simulink model "HarnessModel_CtrlEnv"  (R2026a)
settings: Solver=daessc  StopTime=100  AbsTol=1e-3
PreLoadFcn:
  | setupHarness_CtrlEnv
PostLoadFcn:
  | % Setup the model to use the "Simple" case
  | % for the Vehicle speed reference.
  | loadLUTData_VehSpdRef_Simple
  | set_param(bdroot, StopTime = "100")
  | set_param(bdroot + "/Controller and Environment/Vehicle speed reference", ...
  |     ReferencedSubsystem="VehSpdRef_LookupTable_refsub")
settings Model: Creator=isaacito  LastModifiedBy=isaacito
settings SimscapeCC: SimscapeNominalValues="[{\"value\":\"1\",\"unit\":\"A\"},{\"value\":\"1\",\"unit\":\"bar\"},{\"value\":\"1\",\"unit\":\"cm^2\"},{\"value\":\"1\",\"unit\":\"cm^3/s\"},{\"value\":\"1\",\"unit\":\"kJ/kg\"},{\"value\":\"1\",\"unit\":\"kW\"},{\"value\":\"1\",\"unit\":\"l\"},{\"value\":\"1\",\"unit\":\"N\"},{\"value\":\"1\",\"unit\":\"N*m\"},{\"value\":\"1\",\"unit\":\"V\"}]"  SimscapeLogSimulationStatistics=on  SimscapeLogLimitData=off  SimscapeLogDataHistory=5000.0

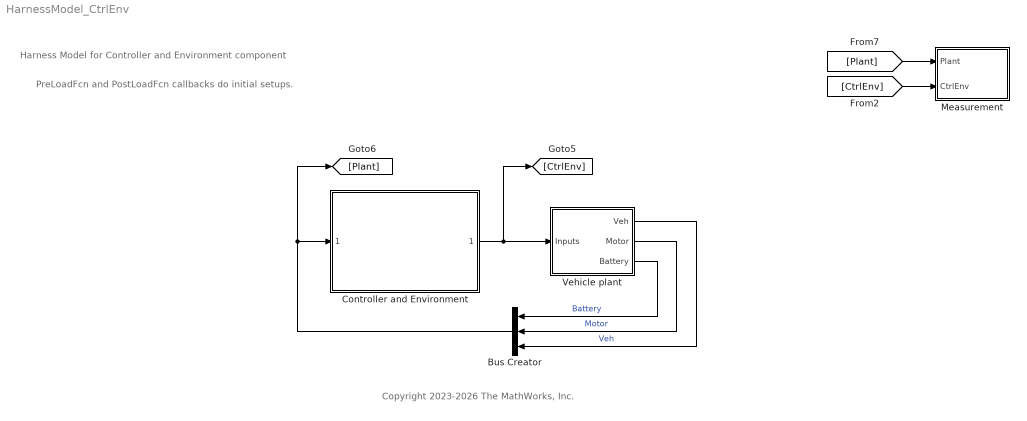
== system HarnessModel_CtrlEnv ==
  note: PreLoadFcn and PostLoadFcn callbacks do initial setups.
  note: Harness Model for Controller and Environment component
  note: Copyright 2023-2026 The MathWorks, Inc.
  Bus Creator : BusCreator  Inputs=3
  Controller and Environment : Subsystem  ReferencedSubsystem=CtrlEnv_Basic_refsub
      settings: OpenFcn=|
      | % Look under mask:
      | open_system(gcb, "force")
  Measurement : Subsystem
  Vehicle plant : Subsystem
  wires:
  [CtrlEnv] -> Measurement/2(CtrlEnv)
  [Plant] -> Measurement/1(Plant)
  Controller and Environment/1 -> Vehicle plant/1(Inputs), [CtrlEnv]
  Vehicle plant/1(Veh) -> Bus Creator/3  "Veh"
  Vehicle plant/2(Motor) -> Bus Creator/2  "Motor"
  Vehicle plant/3(Battery) -> Bus Creator/1  "Battery"
  Bus Creator/1 -> Controller and Environment/1, [Plant]

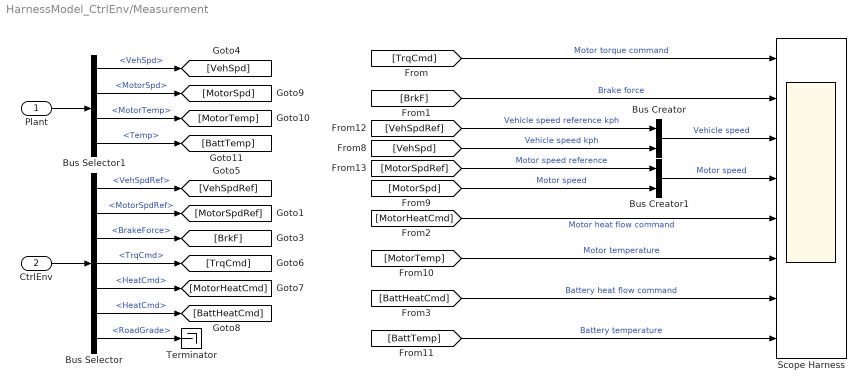
== system HarnessModel_CtrlEnv/Measurement ==
  Plant : Inport
  CtrlEnv : Inport  Port=2
  Bus Creator : BusCreator  Inputs=2
  Bus Creator1 : BusCreator  Inputs=2
  Bus Selector : BusSelector  OutputSignals=Info.VehSpdRef,Info.MotorSpdRef,Vehicle.BrakeForce,MotorDrive.TrqCmd,MotorDrive.HeatCmd,BatteryHV.HeatCmd,Vehicle.RoadGrade
  Bus Selector1 : BusSelector  OutputSignals=Veh.VehSpd,Motor.MotorSpd,Motor.MotorTemp,Battery.Temp
  Scope Harness : Scope  NumInputPorts=8
      settings: ActiveDisplayYMinimum=-87.899049357482824  ActiveDisplayYMaximum=218.53000210473297
  Terminator : Terminator
  wires:
  CtrlEnv/1 -> Bus Selector/1
  Bus Selector/1 -> [VehSpdRef]  "<VehSpdRef>"
  Bus Selector/2 -> [MotorSpdRef]  "<MotorSpdRef>"
  Plant/1 -> Bus Selector1/1
  Bus Selector1/1 -> [VehSpd]  "<VehSpd>"
  Bus Selector1/2 -> [MotorSpd]  "<MotorSpd>"
  Bus Selector1/3 -> [MotorTemp]  "<MotorTemp>"
  Bus Selector1/4 -> [BattTemp]  "<Temp>"
  [VehSpdRef] -> Bus Creator/1  "Vehicle speed reference kph"
  [VehSpd] -> Bus Creator/2  "Vehicle speed kph"
  [MotorSpdRef] -> Bus Creator1/1  "Motor speed reference"
  [MotorSpd] -> Bus Creator1/2  "Motor speed"
  Bus Selector/3 -> [BrkF]  "<BrakeForce>"
  Bus Selector/4 -> [TrqCmd]  "<TrqCmd>"
  Bus Selector/5 -> [MotorHeatCmd]  "<HeatCmd>"
  Bus Selector/6 -> [BattHeatCmd]  "<HeatCmd>"
  Bus Selector/7 -> Terminator/1  "<RoadGrade>"
  [TrqCmd] -> Scope Harness/1  "Motor torque command"
  [BrkF] -> Scope Harness/2  "Brake force"
  Bus Creator/1 -> Scope Harness/3  "Vehicle speed"
  Bus Creator1/1 -> Scope Harness/4  "Motor speed"
  [MotorHeatCmd] -> Scope Harness/5  "Motor heat flow command"
  [MotorTemp] -> Scope Harness/6  "Motor temperature"
  [BattHeatCmd] -> Scope Harness/7  "Battery heat flow command"
  [BattTemp] -> Scope Harness/8  "Battery temperature"

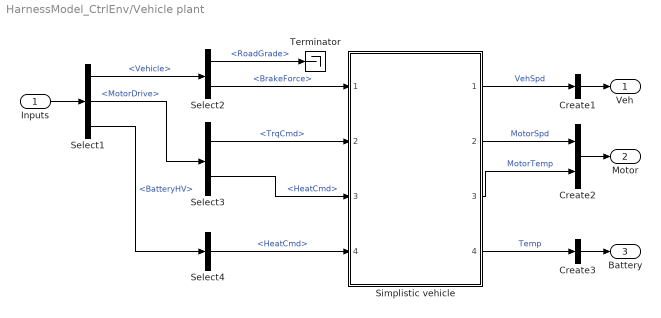
== system HarnessModel_CtrlEnv/Vehicle plant ==
  Inputs : Inport
  Create1 : BusCreator  Inputs=1
  Create2 : BusCreator  Inputs=2
  Create3 : BusCreator  Inputs=1
  Select1 : BusSelector  OutputSignals=Vehicle,MotorDrive,BatteryHV
  Select2 : BusSelector  OutputSignals=RoadGrade,BrakeForce
  Select3 : BusSelector  OutputSignals=TrqCmd,HeatCmd
  Select4 : BusSelector  OutputSignals=HeatCmd
  Simplistic vehicle : Subsystem  ReferencedSubsystem=CtrlEnv_Vehicle_refsub
      settings: OpenFcn="open_system(gcb, \"force\")"
  Terminator : Terminator
  Veh : Outport
  Motor : Outport  Port=2
  Battery : Outport  Port=3
  wires:
  Inputs/1 -> Select1/1
  Select1/1 -> Select2/1  "<Vehicle>"
  Select1/2 -> Select3/1  "<MotorDrive>"
  Select1/3 -> Select4/1  "<BatteryHV>"
  Select2/1 -> Terminator/1  "<RoadGrade>"
  Select2/2 -> Simplistic vehicle/1  "<BrakeForce>"
  Select3/1 -> Simplistic vehicle/2  "<TrqCmd>"
  Select3/2 -> Simplistic vehicle/3  "<HeatCmd>"
  Select4/1 -> Simplistic vehicle/4  "<HeatCmd>"
  Simplistic vehicle/1 -> Create1/1  "VehSpd"
  Create1/1 -> Veh/1
  Simplistic vehicle/2 -> Create2/1  "MotorSpd"
  Create2/1 -> Motor/1
  Create3/1 -> Battery/1
  Simplistic vehicle/4 -> Create3/1  "Temp"
  Simplistic vehicle/3 -> Create2/2  "MotorTemp"
